simulink library "lib_Grid_DC_Static"  (R2026a)
settings: Solver=VariableStepAuto
undefined symbols (not defined in the file): DC, iconductance_matrix
settings Model: Creator=atomas  LastModifiedBy=atomas

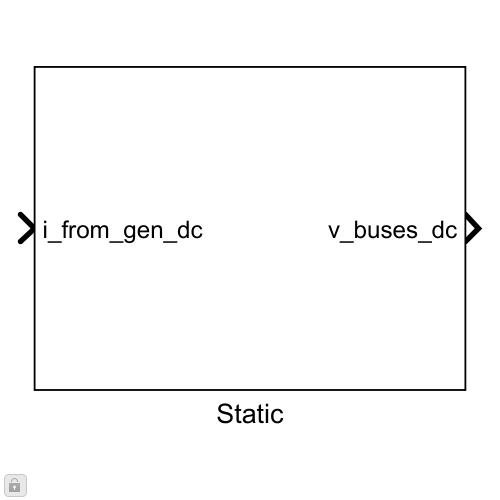
[thumbnail: Simulink's stored preview of the top-level diagram]
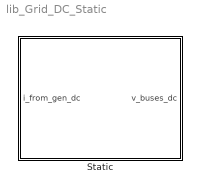
== system lib_Grid_DC_Static ==
  Static : Subsystem  VariantControl=Static

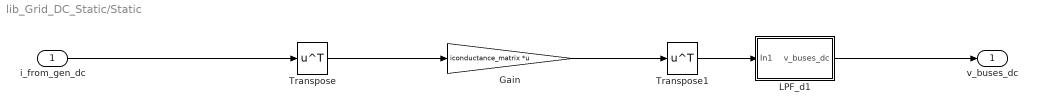
== system lib_Grid_DC_Static/Static ==
  i_from_gen_dc : Inport
  Gain : Gain  Gain=iconductance_matrix  Multiplication=Matrix(K*u)
  LPF_d1 : Subsystem
  Transpose : Math  Operator=transpose
  Transpose1 : Math  Operator=transpose
  v_buses_dc : Outport
  wires:
  Gain/1 -> Transpose1/1
  LPF_d1/1(v_buses_dc) -> v_buses_dc/1
  Transpose1/1 -> LPF_d1/1(In1)
  Transpose/1 -> Gain/1
  i_from_gen_dc/1 -> Transpose/1

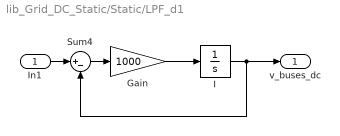
== system lib_Grid_DC_Static/Static/LPF_d1 ==
  In1 : Inport
  Gain : Gain  Gain=1000
  I : Integrator  InitialCondition=DC.v
  Sum4 : Sum  Inputs=|+-
  v_buses_dc : Outport
  wires:
  Sum4/1 -> Gain/1
  In1/1 -> Sum4/1
  I/1 -> v_buses_dc/1, Sum4/2
  Gain/1 -> I/1
